simulink model "GlassAndChamber"  (R2025a)
settings: Solver=VariableStepAuto  StartTime=0.0  StopTime=4000.0  RelTol=1e-3
libraries: simulink x1
settings Model: Creator=Laurenpearse  LastModifiedBy=Laurenpearse

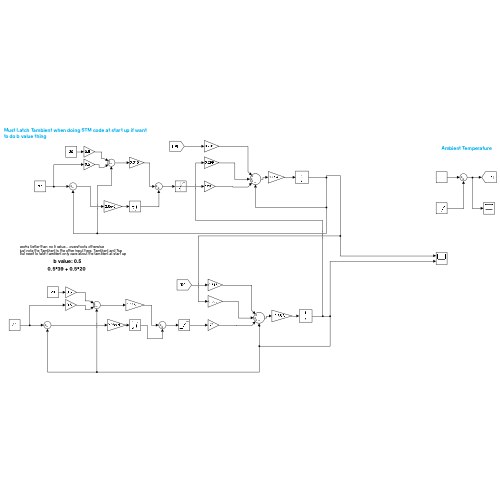
[thumbnail: Simulink's stored preview of the top-level diagram]
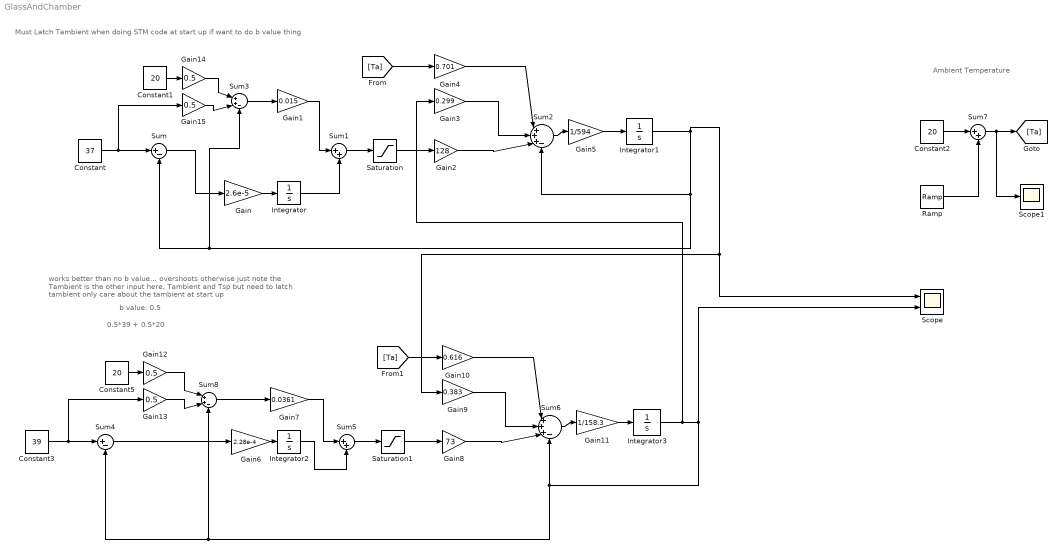
== system GlassAndChamber ==
  note: Ambient Temperature
  note: b value: 0.5
  note: works better than no b value... overshoots otherwise
      | just note the Tambient is the other input here, Tambient and Tsp
      | but need to latch tambient only care about the tambient at start up
  note: 0.5*39 + 0.5*20
  note: Must Latch Tambient when doing STM code at start up if want to do b value thing
  Constant : Constant  Value=37
  Constant1 : Constant  Value=20
  Constant2 : Constant  Value=20
  Constant3 : Constant  Value=39
  Constant5 : Constant  Value=20
  Gain : Gain  Gain=2.6e-5
  Gain1 : Gain  Gain=0.015
  Gain10 : Gain  Gain=0.616
  Gain11 : Gain  Gain=1/158.3
  Gain{12..15} (4 alike) : Gain  Gain=0.5
  Gain2 : Gain  Gain=128
  Gain3 : Gain  Gain=0.299
  Gain4 : Gain  Gain=0.701
  Gain5 : Gain  Gain=1/594
  Gain6 : Gain  Gain=2.28e-4
  Gain7 : Gain  Gain=0.0361
  Gain8 : Gain  Gain=73
  Gain9 : Gain  Gain=0.383
  Integrator : Integrator  LimitOutput=on  UpperSaturationLimit=1  LowerSaturationLimit=0
  Integrator1 : Integrator  InitialCondition=20
  Integrator2 : Integrator  LimitOutput=on  UpperSaturationLimit=1  LowerSaturationLimit=0
  Integrator3 : Integrator  InitialCondition=20
  Ramp : simulink/Sources/Ramp  slope=-0.001  start=0  InitialOutput=0
  Saturation : Saturate  UpperLimit=1  LowerLimit=0
  Saturation1 : Saturate  UpperLimit=1  LowerLimit=0
  Scope : Scope  NumInputPorts=2
      settings: ActiveDisplayYMinimum=40.844588693970536  ActiveDisplayYMaximum=44.663087858876345
  Scope1 : Scope
      settings: ActiveDisplayYMinimum=15.5  ActiveDisplayYMaximum=20.5
  Sum : Sum  Inputs=|+-
  Sum1 : Sum  Inputs=|++
  Sum2 : Sum  Inputs=|+++-
  Sum3 : Sum  Inputs=|++-
  Sum4 : Sum  Inputs=|+-
  Sum5 : Sum  Inputs=|++
  Sum6 : Sum  Inputs=|+++-
  Sum7 : Sum  Inputs=|++
  Sum8 : Sum  Inputs=|++-
  wires:
  Sum/1 -> Gain/1
  Sum2/1 -> Gain5/1
  Gain4/1 -> Sum2/1
  Saturation/1 -> Gain2/1
  Gain5/1 -> Integrator1/1
  Integrator/1 -> Sum1/2
  Gain2/1 -> Sum2/3
  Gain/1 -> Integrator/1
  Gain1/1 -> Sum1/1
  Sum1/1 -> Saturation/1
  Gain3/1 -> Sum2/2
  [Ta] -> Gain4/1
  Gain9/1 -> Sum6/2
  Sum6/1 -> Gain11/1
  Sum5/1 -> Saturation1/1
  Gain7/1 -> Sum5/1
  Gain6/1 -> Integrator2/1
  Integrator3/1 -> Gain3/1, Sum6/4, Sum8/3, Sum4/2, Scope/2
  Integrator2/1 -> Sum5/2
  Constant3/1 -> Gain13/1, Sum4/1
  Saturation1/1 -> Gain8/1
  Gain10/1 -> Sum6/1
  Gain8/1 -> Sum6/3
  Sum4/1 -> Gain6/1
  Gain11/1 -> Integrator3/1
  Sum8/1 -> Gain7/1
  [Ta] -> Gain10/1
  Constant5/1 -> Gain12/1
  Gain12/1 -> Sum8/1
  Gain13/1 -> Sum8/2
  Gain14/1 -> Sum3/1
  Integrator1/1 -> Sum2/4, Sum3/3, Sum/2, Gain9/1, Scope/1
  Constant/1 -> Gain15/1, Sum/1
  Constant1/1 -> Gain14/1
  Gain15/1 -> Sum3/2
  Sum3/1 -> Gain1/1
  Constant2/1 -> Sum7/1
  Ramp/1 -> Sum7/2
  Sum7/1 -> Scope1/1, [Ta]
